simulink model "FMT_M7_FrameQuantizer"  (R2026b)
settings: Solver=FixedStepDiscrete  StopTime=2
settings Model: DataDictionary=Flight_Parameters.sldd  Creator=26718  LastModifiedBy=26718

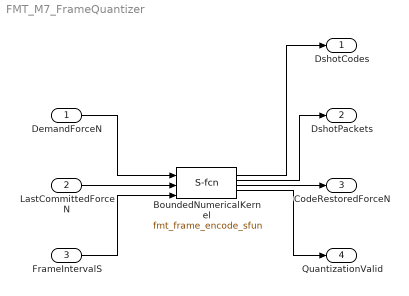
== system FMT_M7_FrameQuantizer ==
  DemandForceN : Inport  OutDataTypeStr=double  PortDimensions=4
  LastCommittedForceN : Inport  Port=2  OutDataTypeStr=double  PortDimensions=4
  FrameIntervalS : Inport  Port=3  OutDataTypeStr=double  PortDimensions=1
  BoundedNumericalKernel : S-Function  FunctionName=fmt_frame_encode_sfun  Parameters=FrameQuantizerParameters  SFunctionDeploymentMode=off  EnableBusSupport=off
  DshotCodes : Outport
  DshotPackets : Outport  Port=2
  CodeRestoredForceN : Outport  Port=3
  QuantizationValid : Outport  Port=4
  wires:
  BoundedNumericalKernel/4 -> QuantizationValid/1
  BoundedNumericalKernel/3 -> CodeRestoredForceN/1
  BoundedNumericalKernel/2 -> DshotPackets/1
  BoundedNumericalKernel/1 -> DshotCodes/1
  FrameIntervalS/1 -> BoundedNumericalKernel/3
  LastCommittedForceN/1 -> BoundedNumericalKernel/2
  DemandForceN/1 -> BoundedNumericalKernel/1
